simulink model "ModelSilnika_MiI2012"  (R2024b)
settings: Solver=FixedStepAuto  StartTime=0.0  StopTime=200  FixedStep=0.01  RelTol=1e-3  EnableMultiTasking=on
libraries: SignalEditorBlockLib x2, fuzblock x1
settings Model: Creator=Milo  LastModifiedBy=Milo
settings SolverCC: AlgebraicLoopSolver=TrustRegion
settings DataIOCC: LimitDataPoints=on  SaveFormat=Array  SignalLoggingSaveFormat=ModelDataLogs  ReturnWorkspaceOutputs=off
settings OptimizationCC: InitFltsAndDblsToZero=on  LifeSpan=inf
settings DebuggingCC: SaveWithParameterizedLinksMsg=none  UnderspecifiedInitializationDetection=Classic  MergeDetectMultiDrivingBlocksExec=none  SignalResolutionControl=TryResolveAllWithWarning  SolverPrmCheckMsg=warning  MultiTaskDSMMsg=warning  MultiTaskCondExecSysMsg=none  FcnCallInpInsideContextMsg=warning  UnconnectedInputMsg=warning  UnconnectedOutputMsg=warning  UnconnectedLineMsg=warning  SFUnexpectedBacktrackingDiag=warning  SFNoUnconditionalDefaultTransitionDiag=warning  SFExecutionAtInitializationDiag=none  ArithmeticOperatorsInVariantConditions=warning
settings HardwareCC: ProdBitPerPointer=32  ProdBitPerSizeT=32  ProdBitPerPtrDiffT=32  ProdLargestAtomicFloat=None  ProdIntDivRoundTo=Undefined  ProdEndianess=Unspecified  ProdWordSize=32  ProdHWDeviceType=32-bit Generic
settings ModelReferenceCC: PropagateSignalLabelsOutOfModel=off
settings RTWCC: GPUComputeCapability=3.5
settings CodeAppCC: StateflowObjectComments=on
settings GRTTargetCC: TargetFcnLib=ansi_tfl_tmw.mat  TargetLangStandard=C89/C90 (ANSI)  CombineOutputUpdateFcns=off  GRTInterface=on
settings ConfigComp: CovMetricSettings=dw  CovSaveCumulativeToWorkspaceVar=on  CovSaveSingleToWorkspaceVar=on

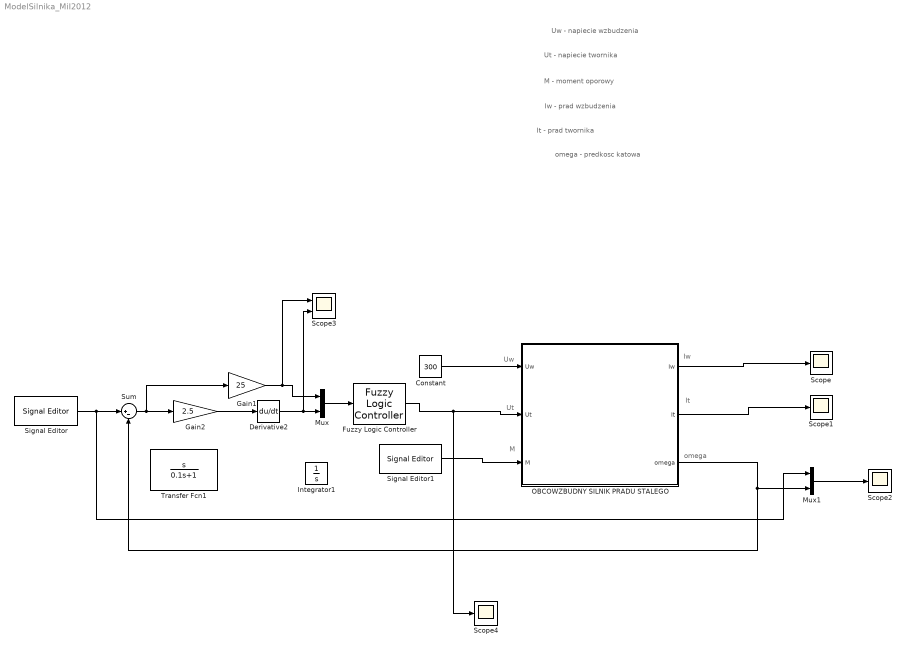
== system ModelSilnika_MiI2012 ==
  note: Uw
  note: Ut
  note: M
  note: Iw
  note: It
  note: omega
  note: Uw - napiecie wzbudzenia
  note: Ut - napiecie twornika
  note: M - moment oporowy
  note: Iw - prad wzbudzenia
  note: It - prad twornika
  note: omega - predkosc katowa
  Constant : Constant  Value=300
  Derivative2 : Derivative
  Fuzzy Logic Controller : fuzblock/Fuzzy Logic  Controller  FIS=silnik_fis  OutputSampleNumber=101  DataType=double  FuzzifiedInputs=off  RuleFiringStrengths=off  RuleOutputs=off  AggregatedOutputs=off  SimulateUsing=Interpreted execution  OutOfRangeInputValueMessage=warning  NoRuleFiredMessage=warning  EmptyOutputFuzzySetMessage=warning
  Gain1 : Gain  Gain=25
  Gain2 : Gain  Gain=2.5
  Integrator1 : Integrator  LimitOutput=on  UpperSaturationLimit=15  LowerSaturationLimit=-15
  Mux : Mux  Inputs=2
  Mux1 : Mux  Inputs=2
  OBCOWZBUDNY SILNIK PRADU STALEGO : Subsystem
      mask init:
      | [data, map]=imread('silnik.gif');
      | pic=ind2rgb(data,map);
      mask Display: image(pic)
  Scope{,1..2,4} (4 alike) : Scope
  Scope3 : Scope  NumInputPorts=2
  Signal Editor : SignalEditorBlockLib/Signal Editor  FileName=Wzad.mat  ActiveScenario=Scenario  ActiveSignal=Signal 1  IsBus=off  OutputBusObjectStr=Bus: BusObject  SampleTime=0.01  ZeroCross=off  OutputAfterFinalValue=Holding final value  Unit=inherit  PreserveSignalName=on  ApplySigPropsToAllScenarios=on  ApplySigPropsToAllSignals=off
  Signal Editor1 : SignalEditorBlockLib/Signal Editor  FileName=M.mat  ActiveScenario=Scenario  ActiveSignal=Signal 1  IsBus=off  OutputBusObjectStr=Bus: BusObject  SampleTime=0.01  ZeroCross=off  OutputAfterFinalValue=Holding final value  Unit=inherit  PreserveSignalName=on  ApplySigPropsToAllScenarios=on  ApplySigPropsToAllSignals=off
  Sum : Sum  Inputs=|+-
  Transfer Fcn1 : TransferFcn  Numerator=[1 0]  Denominator=[0.1 1]
  wires:
  Signal Editor1/1 -> OBCOWZBUDNY SILNIK PRADU STALEGO/3(M)
  Constant/1 -> OBCOWZBUDNY SILNIK PRADU STALEGO/1(Uw)
  Signal Editor/1 -> Mux1/1, Sum/1
  OBCOWZBUDNY SILNIK PRADU STALEGO/3(omega) -> Mux1/2, Sum/2
  Sum/1 -> Gain2/1, Gain1/1
  Mux/1 -> Fuzzy Logic Controller/1
  OBCOWZBUDNY SILNIK PRADU STALEGO/1(Iw) -> Scope/1
  OBCOWZBUDNY SILNIK PRADU STALEGO/2(It) -> Scope1/1
  Mux1/1 -> Scope2/1
  Derivative2/1 -> Scope3/2, Mux/2
  Gain1/1 -> Scope3/1, Mux/1
  Fuzzy Logic Controller/1 -> OBCOWZBUDNY SILNIK PRADU STALEGO/2(Ut), Scope4/1
  Gain2/1 -> Derivative2/1

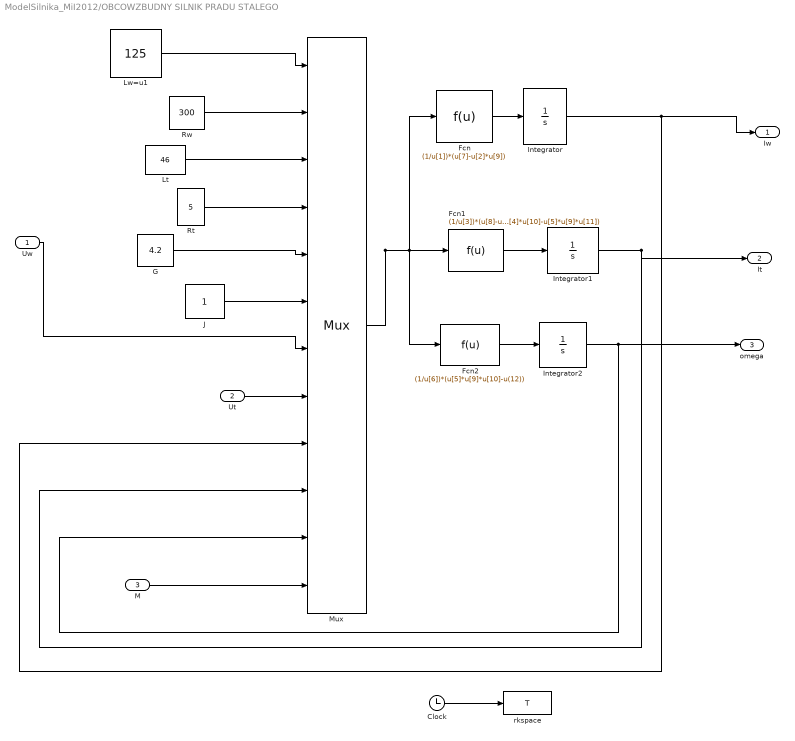
== system ModelSilnika_MiI2012/OBCOWZBUDNY SILNIK PRADU STALEGO ==
  Uw : Inport
  Ut : Inport  Port=2
  M : Inport  Port=3
  Clock : Clock
  Fcn : Fcn  Expr=(1/u[1])*(u[7]-u[2]*u[9])
  Fcn1 : Fcn  Expr=(1/u[3])*(u[8]-u[4]*u[10]-u[5]*u[9]*u[11])
  Fcn2 : Fcn  Expr=(1/u[6])*(u[5]*u[9]*u[10]-u(12))
  G : Constant  Value=4.2
  Integrator : Integrator
  Integrator1 : Integrator
  Integrator2 : Integrator
  J : Constant
  Lt : Constant  Value=46
  Lw=u1 : Constant  Value=125
  Mux : Mux  Inputs=12
  Rt : Constant  Value=5
  Rw : Constant  Value=300
  rkspace : ToWorkspace  VariableName=T  SampleTime=-1
  Iw : Outport
  It : Outport  Port=2
  omega : Outport  Port=3
  wires:
  Lw=u1/1 -> Mux/1
  Rw/1 -> Mux/2
  Lt/1 -> Mux/3
  J/1 -> Mux/6
  Fcn/1 -> Integrator/1
  Fcn1/1 -> Integrator1/1
  Rt/1 -> Mux/4
  Integrator/1 -> Mux/9, Iw/1
  Integrator1/1 -> Mux/10, It/1
  Fcn2/1 -> Integrator2/1
  Integrator2/1 -> Mux/11, omega/1
  Mux/1 -> Fcn/1, Fcn1/1, Fcn2/1
  G/1 -> Mux/5
  Clock/1 -> rkspace/1
  Uw/1 -> Mux/7
  M/1 -> Mux/12
  Ut/1 -> Mux/8
